simulink library "sf_aircraft_lib"  (R2025b)
settings: Solver=VariableStepAuto  StartTime=0.0  StopTime=10.0  RelTol=1e-3
PreLoadFcn:
  | noise_factor=1;
undefined symbols (not defined in the file or in its folder): DEBOUNCE, MAXDELTA, MAXDIFF, MAXVAL, MINVAL
libraries: sf_aircraft_sensor_lib x3
settings Model: Creator=The MathWorks, Inc.  LastModifiedBy=The MathWorks, Inc.
settings RTWCC: LargeConstantGeneration=WriteOnlyDNNConstantsToDataFiles

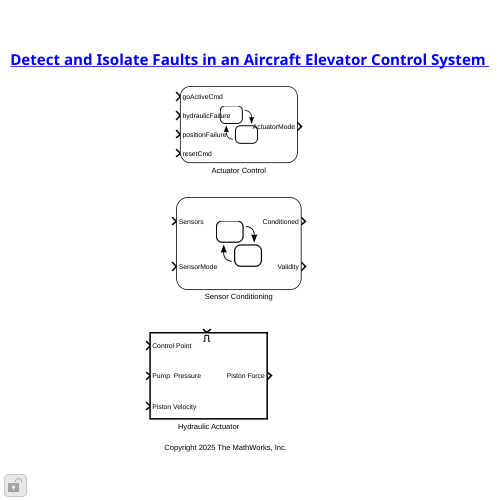
[thumbnail: Simulink's stored preview of the top-level diagram]
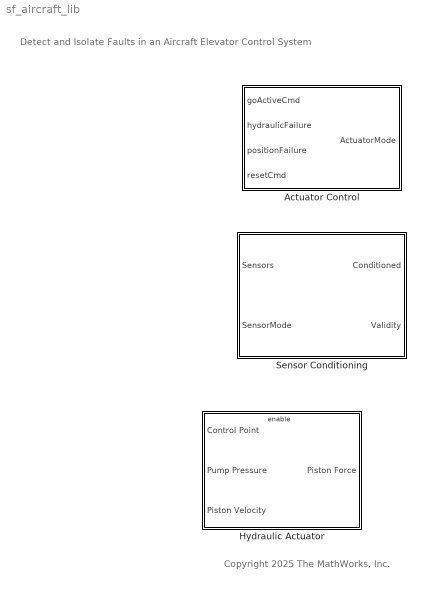
== system sf_aircraft_lib ==
  note: Copyright 2025 The MathWorks, Inc.
  note: Detect and Isolate Faults in an Aircraft Elevator Control System
  Actuator Control : Stateflow chart  TreatAsAtomicUnit=on
  Hydraulic Actuator : Subsystem
  Sensor Conditioning : Stateflow chart  TreatAsAtomicUnit=on

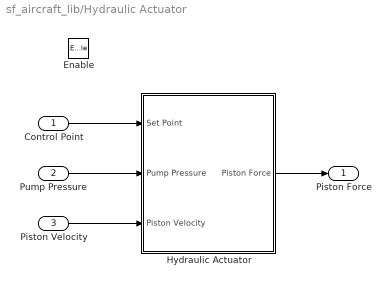
== system sf_aircraft_lib/Hydraulic Actuator ==
  Control Point : Inport
  Pump Pressure : Inport  Port=2
  Piston Velocity : Inport  Port=3
  Enable : EnablePort  StatesWhenEnabling=reset  PropagateVarSize=During execution
  Hydraulic Actuator : Subsystem
  Piston Force : Outport  OutputWhenDisabled=reset  InitialOutput=0  VectorParamsAs1DForOutWhenUnconnected=off
  wires:
  Piston Velocity/1 -> Hydraulic Actuator/3(Piston Velocity)
  Pump Pressure/1 -> Hydraulic Actuator/2(Pump Pressure)
  Control Point/1 -> Hydraulic Actuator/1(Set Point)
  Hydraulic Actuator/1(Piston Force) -> Piston Force/1

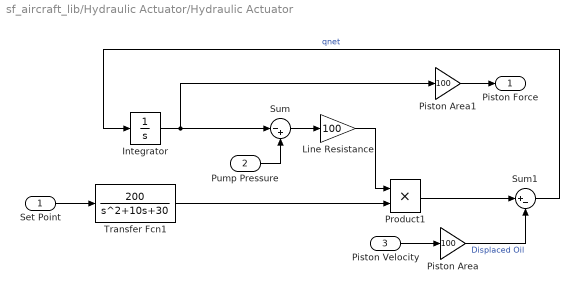
== system sf_aircraft_lib/Hydraulic Actuator/Hydraulic Actuator ==
  Set Point : Inport
  Pump Pressure : Inport  Port=2
  Piston Velocity : Inport  Port=3
  Integrator : Integrator  LimitOutput=on  UpperSaturationLimit=20  LowerSaturationLimit=-20
  Line Resistance : Gain  Gain=100  SaturateOnIntegerOverflow=on  OutDataTypeStr=Inherit: Same as input  ParamDataTypeStr=Inherit: Same as input
  Piston Area : Gain  Gain=100  SaturateOnIntegerOverflow=on  OutDataTypeStr=Inherit: Same as input  ParamDataTypeStr=Inherit: Same as input
  Piston Area1 : Gain  Gain=100  SaturateOnIntegerOverflow=on  OutDataTypeStr=Inherit: Same as input  ParamDataTypeStr=Inherit: Same as input
  Product1 : Product  SaturateOnIntegerOverflow=on  OutDataTypeStr=Inherit: Same as first input
  Sum : Sum  Inputs=|-+  SaturateOnIntegerOverflow=on
  Sum1 : Sum  Inputs=|+-  SaturateOnIntegerOverflow=on
  Transfer Fcn1 : TransferFcn  Numerator=[200]  Denominator=[1 10 30]
  Piston Force : Outport  VectorParamsAs1DForOutWhenUnconnected=off
  wires:
  Integrator/1 -> Piston Area1/1, Sum/1
  Set Point/1 -> Transfer Fcn1/1
  Piston Area1/1 -> Piston Force/1
  Pump Pressure/1 -> Sum/2
  Sum1/1 -> Integrator/1  "qnet"
  Piston Area/1 -> Sum1/2  "Displaced Oil"
  Piston Velocity/1 -> Piston Area/1
  Product1/1 -> Sum1/1
  Transfer Fcn1/1 -> Product1/2
  Line Resistance/1 -> Product1/1
  Sum/1 -> Line Resistance/1

== stateflow chart sf_aircraft_lib/Actuator Control ==
  state On
    state Active
    state Standby
    (default) -> (junction 8)
    (junction 8) -> (junction 7) [order 1]
    (junction 7) -> Active : [goActiveCmd]
    (junction 8) -> (junction 11) [order 2]
    Standby -> (junction 7) : after(1,sec)
    Active -> (junction 14)
    (junction 14) -> Standby : [~goActiveCmd]
    (junction 11) -> Standby
    51 -> Standby
  state Off
    state Recoverable
      ex: Fails = Fails + 1;
    state Isolated
      en: Fails = 0;
    36 -> Isolated
    Recoverable -> 43 [order 1] : [~hydraulicFailure]
    40 -> Recoverable
    Recoverable -> Isolated [order 2] : [Fails >= 5]
  (default) -> On : {Fails=0;}
  44 -> On
  On -> 42 [order 2] : [hydraulicFailure]
  On -> 37 [order 1] : [positionFailure]
  Off -> 52 : [resetCmd] {Fails=0;}
  data: goActiveCmd input; Fails local; hydraulicFailure input; positionFailure input; resetCmd input; ActuatorMode output Enum: ActuatorModeType

== stateflow chart sf_aircraft_lib/Sensor Conditioning ==
  state Sensor1 [parallel]
    settings: executionOrder=1
  state SensorVoting [parallel]
    en,du:
    Validity = uint8(sum(SensorsValid));
    settings: executionOrder=4
    state ThreeValid
      (default) -> (junction 80) : {
          | Conditioned = median(SensorsScreened);
          | }
    state TwoValid
      (default) -> (junction 82) : {
          | Conditioned = mean(SensorsScreened,'omitmissing');
          | }
    state OneValid
      (default) -> (junction 91) : {
          | Conditioned = mean(SensorsScreened,'omitmissing');
          | }
    state ZeroValid
      (default) -> (junction 77) : {
          | % Error reading, will be ignored by controller because Validity == 0
          | %Conditioned = -999;
          | }
    (default) -> (junction 60)
    SensorVoting -> (junction 60) [order 2]
    (junction 60) -> ThreeValid [order 1] : [Validity == 3]
    (junction 60) -> (junction 65) [order 2]
    (junction 65) -> TwoValid [order 1] : [Validity == 2]
    (junction 65) -> (junction 68) [order 2]
    (junction 68) -> OneValid [order 1] : [Validity == 1]
    (junction 68) -> (junction 72) [order 2]
    SensorVoting -> (junction 72) [order 1] : [SensorMode == ActuatorModeType.Isolated]
        | {Validity = 0;}
    (junction 72) -> ZeroValid
  state Sensor2 [parallel]
    settings: executionOrder=2
  state Sensor3 [parallel]
    settings: executionOrder=3
  data: IsValid function_output; Screened function_output; IsValid function_output; Screened function_output; IsValid function_output; Screened function_output; Sensors input double size=3; MAXVAL parameter double size=1; MINVAL parameter double size=1; DEBOUNCE parameter double size=1; MAXDELTA parameter double size=1; MAXDIFF parameter double size=1; Conditioned output double size=1; SensorsScreened local double size=3 =[0 0 0]'; Validity output uint8 size=1; SensorsValid local uint8 size=3 =[0 0 0]'; SensorMode input
